simulink model "Test_2_RS232"  (Simulink 7.0)
settings: Solver=FixedStepDiscrete  StartTime=0.0  StopTime=10.0  FixedStep=0.001  RelTol=1e-3
libraries: dsPICdrivers x9
settings Model: Creator=stefano  LastModifiedBy=stefano
settings OptimizationCC: OptimizeModelRefInitCode=on  LifeSpan=1
settings HardwareCC: ProdBitPerInt=16  ProdEndianess=LittleEndian  ProdWordSize=16  ProdHWDeviceType=16-bit Generic
settings RTWCC: SystemTargetFile=dspic.tlc  TemplateMakefile=dspic_pic30_gcc.tmf  PostCodeGenCommand=dsPIC_Compile()  Description=Embedded Target for Microchip dsPIC (real-time)  ProcessScript=dspic_make_rtw_hook
settings CodeAppCC: IgnoreCustomStorageClasses=off
settings STFCustomTargetCC: GenFloatMathFcnCalls=ANSI_C  ModelReferenceCompliant=off  IncludeMdlTerminateFcn=off  CombineOutputUpdateFcns=on  SuppressErrorStatus=on  ERTCustomFileBanners=on  SupportContinuousTime=off  SupportNonInlinedSFcns=off  SystemTargetFile=dspic.tlc
settings ERTTargetCC: GenFloatMathFcnCalls=ANSI_C  ModelReferenceCompliant=off  CompOptLevelCompliant=off  IncludeMdlTerminateFcn=off  SuppressErrorStatus=on  ModelStepFunctionPrototypeControlCompliant=off  ExtModeMexFile=noextcomm  InlinedParameterPlacement=NonHierarchical  ERTSrcFileBannerTemplate=dsPIC_code_template.cgt  ERTHdrFileBannerTemplate=dsPIC_code_template.cgt  ERTDataSrcFileTemplate=dsPIC_code_template.cgt  ERTDataHdrFileTemplate=dsPIC_code_template.cgt  ERTCustomFileTemplate=dsPIC_main.tlc
settings CustomProperty: DataType=string  Value=C:\PROGRA~1\MATLAB\R2007b\bin\win32\gmake

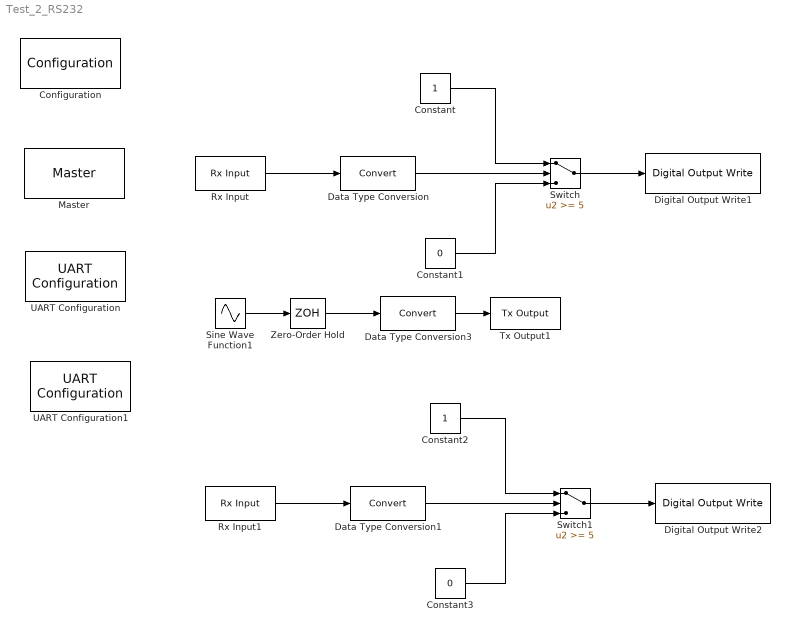
== system Test_2_RS232 ==
  Configuration : dsPICdrivers/Configuration  SystemSampleTime=-1  double64=off
  Constant : Constant  OutDataTypeMode=boolean  OutDataType=sfix(16)  OutScaling=2^0
  Constant1 : Constant  Value=0  OutDataTypeMode=boolean  OutDataType=sfix(16)  OutScaling=2^0
  Constant2 : Constant  OutDataTypeMode=boolean  OutDataType=sfix(16)  OutScaling=2^0
  Constant3 : Constant  Value=0  OutDataTypeMode=boolean  OutDataType=sfix(16)  OutScaling=2^0
  Data Type Conversion : DataTypeConversion  OutDataTypeMode=uint16  OutDataType=sfix(16)  OutScaling=2^0
  Data Type Conversion1 : DataTypeConversion  OutDataTypeMode=uint16  OutDataType=sfix(16)  OutScaling=2^0
  Data Type Conversion3 : DataTypeConversion  OutDataTypeMode=uint8  OutDataType=sfix(16)  OutScaling=2^0
  Digital Output Write1 : dsPICdrivers/Digital I//O/Digital Output Write  Tag=dsPIC_Digital_Output  Priority=5  PORT=B  Pin=[2]  Simultaneous=off  OrderingInOutPopup=None
  Digital Output Write2 : dsPICdrivers/Digital I//O/Digital Output Write  Tag=dsPIC_Digital_Output  Priority=5  PORT=B  Pin=[3]  Simultaneous=off  OrderingInOutPopup=None
  Master : dsPICdrivers/Master  Tag=dsPIC_MASTER  Priority=1  TimeStepType=Timer1  picType=30f3011  fcy=2.5e6  Quartz_33f=5e6  PLLActive_33f=off  fcyDesired_33f=0  tmr1="[1  2499  0]"  tmr1Info="Time Step : 0.001  ;   Error : 0%  PR1=2499"  tmr2345="[0  0  0  0]"  tmr2345cfg=[-1 -1 -1 -1]  IOautoConf=on  typePort="[ 0   0   0   0   0   0   0   0   0   0   0   0   0   0   0   0   0   0  10  10   0   0   0   0   0   0   0   0   0   0   0   0   0   0   0   0   0   0   0   0   0   0   0   0   0   0   4   0   0   0   0   0   0   0   0   0   0   0   0   0   0   0   0   0   0   0   0   0   0   0   0   0   0   0   0   0   0   0   0   0   0   0   0   0   4   5   0   0   0   0   0   0   0   0   0   0   0   0   0   0   0   0   0   0   0   0   0   0   0   0   0   0 ]"  TRIS="[ 65535  65523  65535  65535  65535  65535  65535 ]"  ADPCFG=12  MasterBusyPort=None  MasterOverloadPort=None  FOSC=HS  TempProtection_33f=TEMP_ON  FPBOR=PBOR_OFF  PWRT=PWRT_OFF  MCLR=MCLR_DIS  PowerSave=off
  Rx Input : dsPICdrivers/Serial PORT/Rx Input  Tag=dsPIC_RX  Priority=5  UART=2  SampleTime=-1  BlockingFctChk=off  OutputDefault=0  IsPresentFlagChk=off
  Rx Input1 : dsPICdrivers/Serial PORT/Rx Input  Tag=dsPIC_RX  Priority=5  UART=1  SampleTime=-1  BlockingFctChk=off  OutputDefault=0  IsPresentFlagChk=off
  Sine Wave Function1 : Sin  Amplitude=10  Bias=10
  Switch : Switch  Threshold=5  OutDataType=sfix(16)  OutScaling=2^0
  Switch1 : Switch  Threshold=5  OutDataType=sfix(16)  OutScaling=2^0
  Tx Output1 : dsPICdrivers/Serial PORT/Tx Output  Tag=dsPIC_TX  Priority=5  UART=2  OrderingInOutPopup=None
  UART Configuration : dsPICdrivers/Serial PORT/UART Configuration  Tag=dsPIC_config_UART  Priority=2  UART=2  proposed_BAUD=9600  ALT_TX_RX=on  InterruptTxWhen=When Transmit Buffer is empty  TXInterruptPri=1  TxBufferSize=32  TXEN=on  InterruptRxWhen=When Receive Buffer is full (contain 4 characters)  RXInterruptPri=2  RxBufferSize=32  BAUD=9600  UxBRG=15  Info="UxBRG = 15   ||  Real Baud : 9766   ||  % error : 1.7253  ||  max 0.97656 Bytes / Step"  RealBaud=0
  UART Configuration1 : dsPICdrivers/Serial PORT/UART Configuration  Tag=dsPIC_config_UART  Priority=2  UART=1  proposed_BAUD=9600  ALT_TX_RX=on  InterruptTxWhen=When Transmit Buffer is empty  TXInterruptPri=3  TxBufferSize=32  TXEN=off  InterruptRxWhen=When Receive Buffer is 3/4 full (contain 3 characters)  RXInterruptPri=4  RxBufferSize=32  BAUD=9600  UxBRG=15  Info="UxBRG = 15   ||  Real Baud : 9766   ||  % error : 1.7253  ||  max 0.97656 Bytes / Step"  RealBaud=0
  Zero-Order Hold : ZeroOrderHold  SampleTime=0.05
  wires:
  Rx Input1/1 -> Data Type Conversion1/1
  Data Type Conversion1/1 -> Switch1/2
  Switch1/1 -> Digital Output Write2/1
  Constant3/1 -> Switch1/3
  Constant2/1 -> Switch1/1
  Rx Input/1 -> Data Type Conversion/1
  Data Type Conversion/1 -> Switch/2
  Switch/1 -> Digital Output Write1/1
  Constant1/1 -> Switch/3
  Constant/1 -> Switch/1
  Data Type Conversion3/1 -> Tx Output1/1
  Zero-Order Hold/1 -> Data Type Conversion3/1
  Sine Wave Function1/1 -> Zero-Order Hold/1
